simulink model "Q2"  (R2025b)
settings: Solver=VariableStepAuto  StartTime=0.0  StopTime=10.0  MaxStep=1e-3  RelTol=1e-3
settings Model: Creator=dkaze  LastModifiedBy=dkaze

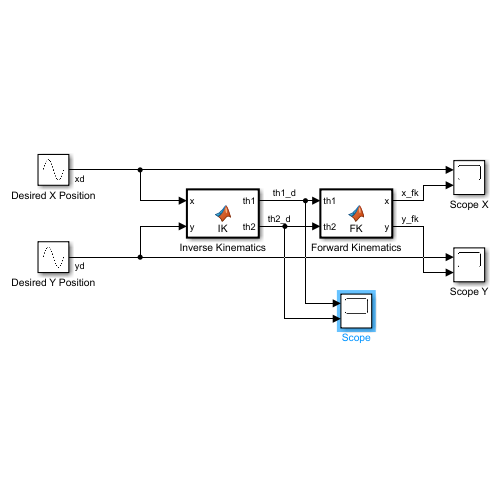
[thumbnail: Simulink's stored preview of the top-level diagram]
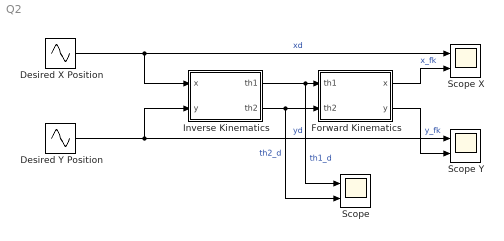
== system Q2 ==
  Desired X Position : Sin  Amplitude=10  Bias=50  Frequency=2*pi/5  Phase=pi/2  SampleTime=0
  Desired Y Position : Sin  Amplitude=10  Bias=20  Frequency=2*pi/5  SampleTime=0
  Forward Kinematics : MATLAB Function  TreatAsAtomicUnit=on
  Inverse Kinematics : MATLAB Function  TreatAsAtomicUnit=on
  Scope : Scope  NumInputPorts=2
      settings: Title=Desired Joint Angle Trajectories  ActiveDisplayYMinimum=-0.73501587548251657  ActiveDisplayYMaximum=2.0967857037729924  YLabel=Joint Angle (rad)
  Scope X : Scope  NumInputPorts=2
      settings: Title=Desired and Reconstructed X Position  ActiveDisplayYMinimum=37.5  ActiveDisplayYMaximum=62.5  YLabel=X Position (cm)
  Scope Y : Scope  NumInputPorts=2
      settings: Title=Desired and Reconstructed Y Position  ActiveDisplayYMinimum=7.4999999999999929  ActiveDisplayYMaximum=32.500000000000007  YLabel=Y Position (cm)  DataLoggingVariableName=ScopeData2
  wires:
  Desired X Position/1 -> Inverse Kinematics/1(x), Scope X/1  "xd"
  Desired Y Position/1 -> Inverse Kinematics/2(y), Scope Y/1  "yd"
  Inverse Kinematics/1(th1) -> Scope/1, Forward Kinematics/1(th1)  "th1_d"
  Inverse Kinematics/2(th2) -> Forward Kinematics/2(th2), Scope/2  "th2_d"
  Forward Kinematics/1(x) -> Scope X/2  "x_fk"
  Forward Kinematics/2(y) -> Scope Y/2  "y_fk"

== matlab function Q2/Inverse Kinematics ==
  data: x input; th1 output; y input; th2 output
function [th1, th2] = IK(x, y)
% Inverse kinematics of 2-DoF planar robot

% Link lengths
L1 = 40;          % cm
L2 = 30;          % cm

% Distance from origin to end-effector
P = sqrt(x^2 + y^2);

% Cosine terms
c1 = (L1^2 + P^2 - L2^2)/(2*L1*P);
c2 = (P^2 - L1^2 - L2^2)/(2*L1*L2);

% Numerical protection
c1 = min(max(c1,-1),1);
c2 = min(max(c2,-1),1);

% Auxiliary angles
b = atan2(y,x);
a = acos(c1);

% Joint angles
th1 = b - a;      %theta1
th2 = acos(c2);   %theta2

end

== matlab function Q2/Forward Kinematics ==
  data: x output; th1 input; y output; th2 input
function [x, y] = FK(th1, th2)
% Forward kinematics of 2-DoF planar robot

% Link lengths
L1 = 40;       % cm
L2 = 30;       % cm

% End-effector position
x = L1*cos(th1) + L2*cos(th1 + th2);
y = L1*sin(th1) + L2*sin(th1 + th2);

end
